simulink model "DWPUSH"  (R2026b)
settings: Solver=VariableStepAuto
undefined symbols (not defined in the file): Ac, Af, Ar, InitLinkage, Left, Linkage, Visual, X, Y, Z
libraries: sm_lib x57, Suspension_Utilities x43, nesl_utility x12, Linkage_Shock x1, fl_lib x1
(part 2 of 4)

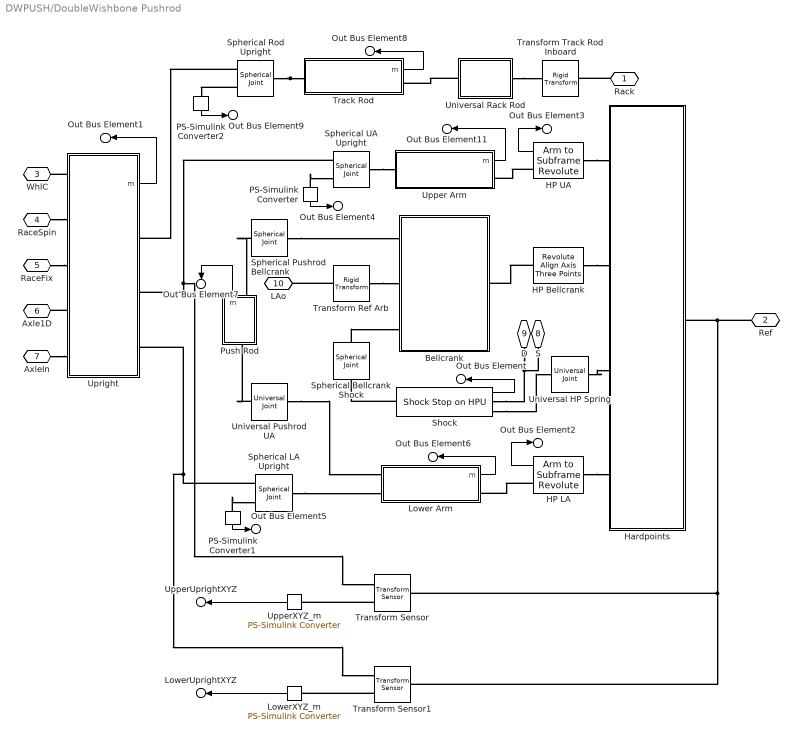
== system DWPUSH/DoubleWishbone Pushrod ==
  Bellcrank : Subsystem  mask(Bellcrank){popup_leftRight=Left, hp_bcr_pivot=hp_bcr_pivot, hp_bcr_shock=hp_spr_bcr, hp_rod=hp_pushrod_in, hp_arb=hp_arb, bcr_mass=bcr_mass, clr_bcr=clr_bcr, opc_bcr=opc_bcr, radius_bcr=radius_bcr}
      mask prompts: popup_leftRight "Left/Right"; hp_bcr_pivot "HP Bellcrank Pivot [xyz] (m)"; hp_bcr_shock "HP Bellcrank Shock [xyz] (m)"; hp_rod "HP Bellcrank Rod [xyz] (m)"; hp_arb "HP Bellcrank ARB [xyz] (m)"; bcr_mass "Mass (kg)"; clr_bcr "Color [RGB]"; opc_bcr "Opacity (0-1)"; radius_bcr "Radius (m)"
      mask help: Models a bellcrank with one pivot and 3 attachment points. The axis of the pivot is normal to the plane formed by the pivot, connection to the rod, and connection to the shock.
      mask init:
      | if(popup_leftRight == 1)
      |     rhs_susp = 1;
      | elseif(popup_leftRight == 2)
      |     rhs_susp = -1;
      | end
      | 
      | rhs_hp = [1 rhs_susp 1];
      mask TypeOptions popup_leftRight: Left | Right
      mask TypeOptions clr_bcr: Arm Pivot ARB/clr_solid | Arm Pivot Rod/clr_solid | Arm Pivot Shock/clr_solid | Arm Rod Shock/clr_solid
      mask TypeOptions opc_bcr: Arm Pivot ARB/opc_solid | Arm Pivot Rod/opc_solid | Arm Pivot Shock/opc_solid | Arm Rod Shock/opc_solid
      mask TypeOptions radius_bcr: Arm Pivot ARB/rad_solid | Arm Pivot Rod/rad_solid | Arm Pivot Shock/rad_solid | Arm Rod Shock/rad_solid
      mask DialogControl cont_ua Prompt: UA
      mask DialogControl cont_vis_ua Prompt: Visualization
      mask Display: image('sm_car_vehicle_linkage_bellcrank_IMAGE.png');
  HP Bellcrank : Suspension_Utilities/Revolute Align Axis Three Points  popup_leftRight=Left  hp_1=hp_bcr_pivot  hp_2=hp_pushrod_in  hp_3=hp_spr_bcr  positionTargetSpecify=off  PositionTargetValue=0
      settings: SourceProductName=SmCar - Suspension Utilites
  HP LA : Suspension_Utilities/Arm to Subframe Revolute  VariantControl=Variant1  LabelModeActiveChoice=Bushing_AxRad  popup_leftRight=Left  hp_f=hp_in_f_ua  hp_r=hp_in_r_ua  Connection=Lower_Arm_to_Subframe  VariantLabel=Lower_Arm_to_Subframe.class.Value
      settings: AttributesFormatString=%<ActiveVariant>  SourceProductName=SmCar - Suspension Utilites
  HP UA : Suspension_Utilities/Arm to Subframe Revolute  VariantControl=Variant1  LabelModeActiveChoice=Bushing_AxRad  popup_leftRight=Left  hp_f=hp_in_f_ua  hp_r=hp_in_r_ua  Connection=Upper_Arm_to_Subframe  VariantLabel=Upper_Arm_to_Subframe.class.Value
      settings: AttributesFormatString=%<ActiveVariant>  SourceProductName=SmCar - Suspension Utilites
  Hardpoints : Subsystem  mask{popup_leftRight=Left, hp_in_f_ua=hp_in_f_ua, hp_in_r_ua=hp_in_r_ua, hp_in_f_la=hp_in_f_la, hp_in_r_la=hp_in_r_la, hp_bellcrank=hp_bcr_pivot, hp_spr_top=hp_spr_body, clr_hp=clr_hp, opc_hp=opc_hp, size_hp=size_hp}
      mask prompts: popup_leftRight "Left/Right"; hp_in_f_ua "Upper Arm Front [xyz] (m)"; hp_in_r_ua "Upper Arm Rear [xyz] (m)"; hp_in_f_la "Lower Arm Front [xyz] (m)"; hp_in_r_la "Lower Arm Rear [xyz] (m)"; hp_bellcrank "Bellcrank Pivot [xyz] (m)"; hp_spr_top "Spring [xyz] (m)"
      mask init:
      | % Set parameter for mirroring (+y or -y)
      | if(popup_leftRight == 1)
      |     rhs_susp = 1;    
      | elseif(popup_leftRight == 2)
      |     rhs_susp = -1;
      | end
      | 
      | rhs_hp = [1 rhs_susp 1];
      mask TypeOptions popup_leftRight: Left | Right
      mask TypeOptions clr_hp: Subsystem/Vis HP LAf/GraphicDiffuseColor | Vis HP LAr/GraphicDiffuseColor | Vis HP Spring/GraphicDiffuseColor | Vis HP UAf/GraphicDiffuseColor | Vis HP UAr/GraphicDiffuseColor
      mask TypeOptions opc_hp: Subsystem/Vis HP LAf/GraphicOpacity | Vis HP LAr/GraphicOpacity | Vis HP Spring/GraphicOpacity | Vis HP UAf/GraphicOpacity | Vis HP UAr/GraphicOpacity
      mask DialogControl cont_hp Prompt: Hardpoints
      mask DialogControl cont_vis_hp Prompt: Visualization
      mask DialogControl text_clr_hp Prompt: Color [RGB]
      mask DialogControl text_opc_hp Prompt: Opac. (0-1)
      mask DialogControl text_size_hp Prompt: Size (m)
      mask DialogControl text_hp Prompt: Hardpoints
      mask Display: image('sm_car_vehicle_linkage_dw_pullrod_hp_IMAGE.png');
  Lower Arm : Subsystem  mask(Lower Arm (Wishbone)){popup_leftRight=Left, hp_in_f=hp_in_f_la, hp_in_r=hp_in_r_la, hp_out=hp_out_la, hp_rod=hp_pushrod_out, la_mass=la_mass, clr_solid=clr_la, opc_solid=opc_la, rad_solid=radius_la}
      mask prompts: popup_leftRight "Left/Right"; hp_in_f "Inboard Front [xyz] (m)"; hp_in_r "Inboard Rear [xyz] (m)"; hp_out "Outboard [xyz] (m)"; hp_rod "Rod [xyz] (m)"; la_mass "Mass (kg)"; clr_solid "Color [RGB]"; opc_solid "Opacity (0-1)"; rad_solid "Radius (m)"
      mask help: This subsystem models the lower arm of a wishbone suspension. It can be configured to have one or two attachment points to the chassis. There are connections to the upright and spring.
      mask init:
      | % Set parameter for mirroring (+y or -y)
      | if(popup_leftRight == 1)
      |     rhs_susp = 1;
      | elseif(popup_leftRight == 2)
      |     rhs_susp = -1;
      | end
      | 
      | rhs_hp = [1 rhs_susp 1];
      | 
      | 
      |     hp_rod_f=hp_out-(hp_out-hp_in_f)/2;
      |     hp_rod_r=hp_out-(hp_out-hp_in_r)/2;
      mask Help: web ('sm_car_lower_arm_help.html')
      mask TypeOptions popup_leftRight: Left | Right
      mask TypeOptions clr_solid: Arm F1/clr_solid | Arm F2/clr_solid | Arm R1/clr_solid | Arm R2/clr_solid
      mask TypeOptions opc_solid: Arm F1/opc_solid | Arm F2/opc_solid | Arm R1/opc_solid | Arm R2/opc_solid
      mask TypeOptions rad_solid: Arm F1/rad_solid | Arm F2/rad_solid | Arm R1/rad_solid | Arm R2/rad_solid
      mask DialogControl cont_ua Prompt: LA
      mask DialogControl cont_vis_la Prompt: Visualization
      mask Display: image('sm_car_vehicle_linkage_dw_ua_IMAGE.png');
  LowerXYZ_m : nesl_utility/PS-Simulink Converter  PhysicalDomain=network_engine_domain  SubClassName=ps_output  LeftPortType=input  RightPortType=output  PseudoPeriodic=off  Frequencies=[]  VectorFormat=inherit  Unit=m  AffineConversion=off
  PS-Simulink Converter : nesl_utility/PS-Simulink Converter  PhysicalDomain=network_engine_domain  SubClassName=ps_output  LeftPortType=input  RightPortType=output  PseudoPeriodic=off  Frequencies=[]  VectorFormat=inherit  Unit=inherit  AffineConversion=off
  PS-Simulink Converter1 : nesl_utility/PS-Simulink Converter  PhysicalDomain=network_engine_domain  SubClassName=ps_output  LeftPortType=input  RightPortType=output  PseudoPeriodic=off  Frequencies=[]  VectorFormat=inherit  Unit=inherit  AffineConversion=off
  PS-Simulink Converter2 : nesl_utility/PS-Simulink Converter  PhysicalDomain=network_engine_domain  SubClassName=ps_output  LeftPortType=input  RightPortType=output  PseudoPeriodic=off  Frequencies=[]  VectorFormat=inherit  Unit=inherit  AffineConversion=off
  Push Rod : Subsystem  VariantControl=Steer  mask(Rod){popup_leftRight=Left, hp_in=hp_pushrod_in, hp_out=hp_pushrod_out, rod_mass=pullrod_mass, clr_conn_rod=clr_conn_pullrod, opc_conn_rod=opc_conn_pullrod, size_conn_rod=size_conn_pullrod, clr_rod=clr_pullrod, opc_rod=opc_pullrod, radius_rod=radius_pullrod}
      mask prompts: popup_leftRight "Left/Right"; hp_in "Bellcrank [xyz] (m)"; hp_out "Upper Arm [xyz] (m)"; rod_mass "Mass (Kg)"
      mask help: Rod connecting two hard points
      mask init:
      | if(popup_leftRight == 1)
      |     rhs_rod = 1;
      | elseif(popup_leftRight == 2)
      |     rhs_rod = -1;
      | end
      | rhs_hp=[1 rhs_rod 1];
      | 
      |     hp_rod_c=hp_out-(hp_out-hp_in)/2;
      mask TypeOptions popup_leftRight: Left | Right
      mask TypeOptions clr_conn_rod:
      | Vis
      | Rod
      | Out/GraphicDiffuseColor | Vis
      | Rod
      | In/GraphicDiffuseColor
      mask TypeOptions opc_conn_rod:
      | Vis
      | Rod
      | Out/GraphicOpacity | Vis
      | Rod
      | In/GraphicOpacity
      mask TypeOptions clr_rod: Rod/clr_solid
      mask TypeOptions opc_rod: Rod/opc_solid
      mask TypeOptions radius_rod: Rod/rad_solid
      mask DialogControl cont_rod Prompt: Rod
      mask DialogControl grp_rod Prompt: Rod
      mask DialogControl cont_vis_rod Prompt: Visualization
      mask DialogControl text_clr_rod Prompt: Color [RGB]
      mask DialogControl text_opc_rod Prompt: Opac. (0-1)
      mask DialogControl text_size_rod Prompt: Size (m)
      mask DialogControl text_conn_rod Prompt: Connections
      mask DialogControl text_rod_rod Prompt: Rod
      mask Display: image('sm_car_vehicle_linkage_pushrod_IMAGE.png');
  Shock : Linkage_Shock/Shock Stop on HPU  shock_pist_mass=shock_pist_mass  shock_cyl_mass=shock_cyl_mass  hp_spr_top=hp_spr_body  hp_spr_bot=hp_spr_bcr  up_lim_bumpstop=up_lim_bumpstop  low_lim_bumpstop=low_lim_bumpstop  clr_conn_shock=clr_conn_shock  opc_conn_shock=opc_conn_shock  size_conn_shock=size_conn_shock  clr_shock_cyl=clr_shock_cyl  opc_shock_cyl=opc_shock_cyl  radius_shock_cyl=radius_shock_cyl  clr_shock_piston=clr_shock_piston  opc_shock_piston=opc_shock_piston  clr_shock_bumpstop=clr_shock_bumpstop  opc_shock_bumpstop=opc_shock_bumpstop  deadvol_len_shock_cyl=deadvol_len_shock_cyl  piston_len_shock=piston_len_shock  cyl_cap_len_shock=cyl_cap_len_shock  bumpstop_len_shock=bumpstop_len_shock
  Spherical Bellcrank Shock : sm_lib/Joints/Spherical Joint  JointMode=Normal  CompositeWrenchDir=FollowerOnBase  CompositeWrenchFrame=BaseFrame  SenseConstraintForce=off  SenseConstraintTorque=off  SenseTotalForce=off  SenseTotalTorque=off  PositionTargetSpecify=off  PositionTargetPriority=High  PositionTargetRotationMethod=None  PositionTargetFollAlignAxisA=+X  PositionTargetBaseAlignAxisA=+Y  PositionTargetFollAlignAxisB=+Y  PositionTargetBaseAlignAxisB=+Z  PositionTargetRotationStandardAxis=+Z  PositionTargetRotationAngle=0.0  PositionTargetRotationAngleUnits=deg  PositionTargetRotationArbitraryAxis=[0 0 1]  PositionTargetRotationSequenceAxes=FollowerAxes  PositionTargetRotationSequence=XYX  PositionTargetRotationSequenceAngles=[0 0 0]  PositionTargetRotationSequenceAnglesUnits=deg  PositionTargetRotationMatrix=[1 0 0; 0 1 0; 0 0 1]  PositionTargetQuaternion=[1 0 0 0]  VelocityTargetSpecify=off  VelocityTargetPriority=High  VelocityTargetValue=[0 0 0]  VelocityTargetValueUnits=deg/s  VelocityTargetInFollowerFrame=on  EqPosRotationMethod=None  EqPosFollAlignAxisA=+X  EqPosBaseAlignAxisA=+Y  EqPosFollAlignAxisB=+Y  EqPosBaseAlignAxisB=+Z  EqPosRotationStandardAxis=+Z  EqPosRotationAngle=0.0  EqPosRotationAngleUnits=deg  EqPosRotationArbitraryAxis=[0 0 1]  EqPosRotationSequenceAxes=FollowerAxes  EqPosRotationSequence=XYX  EqPosRotationSequenceAngles=[0 0 0]  EqPosRotationSequenceAnglesUnits=deg  EqPosRotationMatrix=[1 0 0; 0 1 0; 0 0 1]  EqPosQuaternion=[1 0 0 0]  SpringStiffness=0  SpringStiffnessUnits=N*m/deg  DampingCoefficient=0  DampingCoefficientUnits=N*m/(deg/s)  LowerLimitSpecify=off  LowerLimitBound=15  LowerLimitBoundUnits=deg  LowerLimitStiffness=1e4  LowerLimitStiffnessUnits=N*m/deg  LowerLimitDamping=10  LowerLimitDampingUnits=N*m/(deg/s)  LowerLimitTransitionRegionWidth=0.1  LowerLimitTransitionRegionWidthUnits=deg  UpperLimitSpecify=off  UpperLimitBound=45  UpperLimitBoundUnits=deg  UpperLimitStiffness=1e4  UpperLimitStiffnessUnits=N*m/deg  UpperLimitDamping=10  UpperLimitDampingUnits=N*m/(deg/s)  UpperLimitTransitionRegionWidth=0.1  UpperLimitTransitionRegionWidthUnits=deg  TorqueActuationMode=NoTorque  ActuateTorqueX=off  ActuateTorqueY=off  ActuateTorqueZ=off  ActuateTorque=off  ActuationFrame=BaseFrame  SensePosition=off  SenseVelocityX=off  SenseVelocityY=off  SenseVelocityZ=off  SenseVelocity=off  SenseAccelerationX=off  SenseAccelerationY=off  SenseAccelerationZ=off  SenseAcceleration=off  SenseLowerLimitTorqueMag=off  SenseUpperLimitTorqueMag=off  SensingFrame=BaseFrame
  Spherical LA Upright : sm_lib/Joints/Spherical Joint  JointMode=Normal  CompositeWrenchDir=FollowerOnBase  CompositeWrenchFrame=BaseFrame  SenseConstraintForce=off  SenseConstraintTorque=off  SenseTotalForce=on  SenseTotalTorque=off  PositionTargetSpecify=off  PositionTargetPriority=High  PositionTargetRotationMethod=None  PositionTargetFollAlignAxisA=+X  PositionTargetBaseAlignAxisA=+Y  PositionTargetFollAlignAxisB=+Y  PositionTargetBaseAlignAxisB=+Z  PositionTargetRotationStandardAxis=+Z  PositionTargetRotationAngle=0.0  PositionTargetRotationAngleUnits=deg  PositionTargetRotationArbitraryAxis=[0 0 1]  PositionTargetRotationSequenceAxes=FollowerAxes  PositionTargetRotationSequence=XYX  PositionTargetRotationSequenceAngles=[0 0 0]  PositionTargetRotationSequenceAnglesUnits=deg  PositionTargetRotationMatrix=[1 0 0; 0 1 0; 0 0 1]  PositionTargetQuaternion=[1 0 0 0]  VelocityTargetSpecify=off  VelocityTargetPriority=High  VelocityTargetValue=[0 0 0]  VelocityTargetValueUnits=deg/s  VelocityTargetInFollowerFrame=on  EqPosRotationMethod=None  EqPosFollAlignAxisA=+X  EqPosBaseAlignAxisA=+Y  EqPosFollAlignAxisB=+Y  EqPosBaseAlignAxisB=+Z  EqPosRotationStandardAxis=+Z  EqPosRotationAngle=0.0  EqPosRotationAngleUnits=deg  EqPosRotationArbitraryAxis=[0 0 1]  EqPosRotationSequenceAxes=FollowerAxes  EqPosRotationSequence=XYX  EqPosRotationSequenceAngles=[0 0 0]  EqPosRotationSequenceAnglesUnits=deg  EqPosRotationMatrix=[1 0 0; 0 1 0; 0 0 1]  EqPosQuaternion=[1 0 0 0]  SpringStiffness=0  SpringStiffnessUnits=N*m/deg  DampingCoefficient=0  DampingCoefficientUnits=N*m/(deg/s)  LowerLimitSpecify=off  LowerLimitBound=15  LowerLimitBoundUnits=deg  LowerLimitStiffness=1e4  LowerLimitStiffnessUnits=N*m/deg  LowerLimitDamping=10  LowerLimitDampingUnits=N*m/(deg/s)  LowerLimitTransitionRegionWidth=0.1  LowerLimitTransitionRegionWidthUnits=deg  UpperLimitSpecify=off  UpperLimitBound=45  UpperLimitBoundUnits=deg  UpperLimitStiffness=1e4  UpperLimitStiffnessUnits=N*m/deg  UpperLimitDamping=10  UpperLimitDampingUnits=N*m/(deg/s)  UpperLimitTransitionRegionWidth=0.1  UpperLimitTransitionRegionWidthUnits=deg  TorqueActuationMode=NoTorque  ActuateTorqueX=off  ActuateTorqueY=off  ActuateTorqueZ=off  ActuateTorque=off  ActuationFrame=BaseFrame  SensePosition=off  SenseVelocityX=off  SenseVelocityY=off  SenseVelocityZ=off  SenseVelocity=off  SenseAccelerationX=off  SenseAccelerationY=off  SenseAccelerationZ=off  SenseAcceleration=off  SenseLowerLimitTorqueMag=off  SenseUpperLimitTorqueMag=off  SensingFrame=BaseFrame
  Spherical Pushrod Bellcrank : sm_lib/Joints/Spherical Joint  JointMode=Normal  CompositeWrenchDir=FollowerOnBase  CompositeWrenchFrame=BaseFrame  SenseConstraintForce=off  SenseConstraintTorque=off  SenseTotalForce=off  SenseTotalTorque=off  PositionTargetSpecify=off  PositionTargetPriority=High  PositionTargetRotationMethod=None  PositionTargetFollAlignAxisA=+X  PositionTargetBaseAlignAxisA=+Y  PositionTargetFollAlignAxisB=+Y  PositionTargetBaseAlignAxisB=+Z  PositionTargetRotationStandardAxis=+Z  PositionTargetRotationAngle=0.0  PositionTargetRotationAngleUnits=deg  PositionTargetRotationArbitraryAxis=[0 0 1]  PositionTargetRotationSequenceAxes=FollowerAxes  PositionTargetRotationSequence=XYX  PositionTargetRotationSequenceAngles=[0 0 0]  PositionTargetRotationSequenceAnglesUnits=deg  PositionTargetRotationMatrix=[1 0 0; 0 1 0; 0 0 1]  PositionTargetQuaternion=[1 0 0 0]  VelocityTargetSpecify=off  VelocityTargetPriority=High  VelocityTargetValue=[0 0 0]  VelocityTargetValueUnits=deg/s  VelocityTargetInFollowerFrame=on  EqPosRotationMethod=None  EqPosFollAlignAxisA=+X  EqPosBaseAlignAxisA=+Y  EqPosFollAlignAxisB=+Y  EqPosBaseAlignAxisB=+Z  EqPosRotationStandardAxis=+Z  EqPosRotationAngle=0.0  EqPosRotationAngleUnits=deg  EqPosRotationArbitraryAxis=[0 0 1]  EqPosRotationSequenceAxes=FollowerAxes  EqPosRotationSequence=XYX  EqPosRotationSequenceAngles=[0 0 0]  EqPosRotationSequenceAnglesUnits=deg  EqPosRotationMatrix=[1 0 0; 0 1 0; 0 0 1]  EqPosQuaternion=[1 0 0 0]  SpringStiffness=0  SpringStiffnessUnits=N*m/deg  DampingCoefficient=0  DampingCoefficientUnits=N*m/(deg/s)  LowerLimitSpecify=off  LowerLimitBound=15  LowerLimitBoundUnits=deg  LowerLimitStiffness=1e4  LowerLimitStiffnessUnits=N*m/deg  LowerLimitDamping=10  LowerLimitDampingUnits=N*m/(deg/s)  LowerLimitTransitionRegionWidth=0.1  LowerLimitTransitionRegionWidthUnits=deg  UpperLimitSpecify=off  UpperLimitBound=45  UpperLimitBoundUnits=deg  UpperLimitStiffness=1e4  UpperLimitStiffnessUnits=N*m/deg  UpperLimitDamping=10  UpperLimitDampingUnits=N*m/(deg/s)  UpperLimitTransitionRegionWidth=0.1  UpperLimitTransitionRegionWidthUnits=deg  TorqueActuationMode=NoTorque  ActuateTorqueX=off  ActuateTorqueY=off  ActuateTorqueZ=off  ActuateTorque=off  ActuationFrame=BaseFrame  SensePosition=off  SenseVelocityX=off  SenseVelocityY=off  SenseVelocityZ=off  SenseVelocity=off  SenseAccelerationX=off  SenseAccelerationY=off  SenseAccelerationZ=off  SenseAcceleration=off  SenseLowerLimitTorqueMag=off  SenseUpperLimitTorqueMag=off  SensingFrame=BaseFrame
  Spherical Rod Upright : sm_lib/Joints/Spherical Joint  JointMode=Normal  CompositeWrenchDir=FollowerOnBase  CompositeWrenchFrame=BaseFrame  SenseConstraintForce=off  SenseConstraintTorque=off  SenseTotalForce=on  SenseTotalTorque=off  PositionTargetSpecify=off  PositionTargetPriority=High  PositionTargetRotationMethod=None  PositionTargetFollAlignAxisA=+X  PositionTargetBaseAlignAxisA=+Y  PositionTargetFollAlignAxisB=+Y  PositionTargetBaseAlignAxisB=+Z  PositionTargetRotationStandardAxis=+Z  PositionTargetRotationAngle=0.0  PositionTargetRotationAngleUnits=deg  PositionTargetRotationArbitraryAxis=[0 0 1]  PositionTargetRotationSequenceAxes=FollowerAxes  PositionTargetRotationSequence=XYX  PositionTargetRotationSequenceAngles=[0 0 0]  PositionTargetRotationSequenceAnglesUnits=deg  PositionTargetRotationMatrix=[1 0 0; 0 1 0; 0 0 1]  PositionTargetQuaternion=[1 0 0 0]  VelocityTargetSpecify=off  VelocityTargetPriority=High  VelocityTargetValue=[0 0 0]  VelocityTargetValueUnits=deg/s  VelocityTargetInFollowerFrame=on  EqPosRotationMethod=None  EqPosFollAlignAxisA=+X  EqPosBaseAlignAxisA=+Y  EqPosFollAlignAxisB=+Y  EqPosBaseAlignAxisB=+Z  EqPosRotationStandardAxis=+Z  EqPosRotationAngle=0.0  EqPosRotationAngleUnits=deg  EqPosRotationArbitraryAxis=[0 0 1]  EqPosRotationSequenceAxes=FollowerAxes  EqPosRotationSequence=XYX  EqPosRotationSequenceAngles=[0 0 0]  EqPosRotationSequenceAnglesUnits=deg  EqPosRotationMatrix=[1 0 0; 0 1 0; 0 0 1]  EqPosQuaternion=[1 0 0 0]  SpringStiffness=0  SpringStiffnessUnits=N*m/deg  DampingCoefficient=0  DampingCoefficientUnits=N*m/(deg/s)  LowerLimitSpecify=off  LowerLimitBound=15  LowerLimitBoundUnits=deg  LowerLimitStiffness=1e4  LowerLimitStiffnessUnits=N*m/deg  LowerLimitDamping=10  LowerLimitDampingUnits=N*m/(deg/s)  LowerLimitTransitionRegionWidth=0.1  LowerLimitTransitionRegionWidthUnits=deg  UpperLimitSpecify=off  UpperLimitBound=45  UpperLimitBoundUnits=deg  UpperLimitStiffness=1e4  UpperLimitStiffnessUnits=N*m/deg  UpperLimitDamping=10  UpperLimitDampingUnits=N*m/(deg/s)  UpperLimitTransitionRegionWidth=0.1  UpperLimitTransitionRegionWidthUnits=deg  TorqueActuationMode=NoTorque  ActuateTorqueX=off  ActuateTorqueY=off  ActuateTorqueZ=off  ActuateTorque=off  ActuationFrame=BaseFrame  SensePosition=off  SenseVelocityX=off  SenseVelocityY=off  SenseVelocityZ=off  SenseVelocity=off  SenseAccelerationX=off  SenseAccelerationY=off  SenseAccelerationZ=off  SenseAcceleration=off  SenseLowerLimitTorqueMag=off  SenseUpperLimitTorqueMag=off  SensingFrame=BaseFrame
  Spherical UA Upright : sm_lib/Joints/Spherical Joint  JointMode=Normal  CompositeWrenchDir=FollowerOnBase  CompositeWrenchFrame=BaseFrame  SenseConstraintForce=off  SenseConstraintTorque=off  SenseTotalForce=on  SenseTotalTorque=off  PositionTargetSpecify=on  PositionTargetPriority=High  PositionTargetRotationMethod=StandardAxis  PositionTargetFollAlignAxisA=+X  PositionTargetBaseAlignAxisA=+Y  PositionTargetFollAlignAxisB=+Y  PositionTargetBaseAlignAxisB=+Z  PositionTargetRotationStandardAxis=+Z  PositionTargetRotationAngle=0.0  PositionTargetRotationAngleUnits=deg  PositionTargetRotationArbitraryAxis=[0 0 1]  PositionTargetRotationSequenceAxes=FollowerAxes  PositionTargetRotationSequence=XYX  PositionTargetRotationSequenceAngles=[0 0 0]  PositionTargetRotationSequenceAnglesUnits=deg  PositionTargetRotationMatrix=[1 0 0; 0 1 0; 0 0 1]  PositionTargetQuaternion=[1 0 0 0]  VelocityTargetSpecify=off  VelocityTargetPriority=High  VelocityTargetValue=[0 0 0]  VelocityTargetValueUnits=deg/s  VelocityTargetInFollowerFrame=on  EqPosRotationMethod=None  EqPosFollAlignAxisA=+X  EqPosBaseAlignAxisA=+Y  EqPosFollAlignAxisB=+Y  EqPosBaseAlignAxisB=+Z  EqPosRotationStandardAxis=+Z  EqPosRotationAngle=0.0  EqPosRotationAngleUnits=deg  EqPosRotationArbitraryAxis=[0 0 1]  EqPosRotationSequenceAxes=FollowerAxes  EqPosRotationSequence=XYX  EqPosRotationSequenceAngles=[0 0 0]  EqPosRotationSequenceAnglesUnits=deg  EqPosRotationMatrix=[1 0 0; 0 1 0; 0 0 1]  EqPosQuaternion=[1 0 0 0]  SpringStiffness=0  SpringStiffnessUnits=N*m/deg  DampingCoefficient=0  DampingCoefficientUnits=N*m/(deg/s)  LowerLimitSpecify=off  LowerLimitBound=15  LowerLimitBoundUnits=deg  LowerLimitStiffness=1e4  LowerLimitStiffnessUnits=N*m/deg  LowerLimitDamping=10  LowerLimitDampingUnits=N*m/(deg/s)  LowerLimitTransitionRegionWidth=0.1  LowerLimitTransitionRegionWidthUnits=deg  UpperLimitSpecify=off  UpperLimitBound=45  UpperLimitBoundUnits=deg  UpperLimitStiffness=1e4  UpperLimitStiffnessUnits=N*m/deg  UpperLimitDamping=10  UpperLimitDampingUnits=N*m/(deg/s)  UpperLimitTransitionRegionWidth=0.1  UpperLimitTransitionRegionWidthUnits=deg  TorqueActuationMode=NoTorque  ActuateTorqueX=off  ActuateTorqueY=off  ActuateTorqueZ=off  ActuateTorque=off  ActuationFrame=BaseFrame  SensePosition=off  SenseVelocityX=off  SenseVelocityY=off  SenseVelocityZ=off  SenseVelocity=off  SenseAccelerationX=off  SenseAccelerationY=off  SenseAccelerationZ=off  SenseAcceleration=off  SenseLowerLimitTorqueMag=off  SenseUpperLimitTorqueMag=off  SensingFrame=FollowerFrame
  Track Rod : Subsystem  VariantControl=Steer  mask(Rod){popup_leftRight=Left, hp_in=hp_in_rod, hp_out=hp_upr_rod, rod_mass=rod_mass, clr_conn_rod=clr_conn_rod, opc_conn_rod=opc_conn_rod, size_conn_rod=size_conn_rod, clr_rod=clr_rod, opc_rod=opc_rod, radius_rod=radius_rod}
      mask prompts: popup_leftRight "Left/Right"; hp_in "Inboard [xyz] (m)"; hp_out "Outboard [xyz] (m)"; rod_mass "Mass (kg)"
      mask help: Rod connecting two hard points
      mask init:
      | if(popup_leftRight == 1)
      |     rhs_rod = 1;
      | elseif(popup_leftRight == 2)
      |     rhs_rod = -1;
      | end
      | rhs_hp=[1 rhs_rod 1];
      | hp_rod_c=hp_out-(hp_out-hp_in)/2;
      mask TypeOptions popup_leftRight: Left | Right
      mask TypeOptions rod_mass: Rod/Mass
      mask TypeOptions clr_conn_rod:
      | Vis
      | Upright
      | Steer/GraphicDiffuseColor | Vis
      | Rack
      | Rod/GraphicDiffuseColor
      mask TypeOptions opc_conn_rod:
      | Vis
      | Upright
      | Steer/GraphicOpacity | Vis
      | Rack
      | Rod/GraphicOpacity
      mask TypeOptions clr_rod: Rod/clr_solid
      mask TypeOptions opc_rod: Rod/opc_solid
      mask TypeOptions radius_rod: Rod/rad_solid
      mask DialogControl cont_rod Prompt: Rod
      mask DialogControl grp_rod Prompt: Rod
      mask DialogControl cont_vis_rod Prompt: Visualization
      mask DialogControl text_clr_rod Prompt: Color [RGB]
      mask DialogControl text_opc_rod Prompt: Opac. (0-1)
      mask DialogControl text_size_rod Prompt: Size (m)
      mask DialogControl text_conn_rod Prompt: Connections
      mask DialogControl text_rod_rod Prompt: Rod
      mask Display: image('sm_car_linkage_trackrod_IMAGE.png');
  Transform Ref Arb : sm_lib/Frames and Transforms/Rigid Transform  RotationMethod=None  FollAlignAxisA=+X  BaseAlignAxisA=+Y  FollAlignAxisB=+Y  BaseAlignAxisB=+Z  RotationStandardAxis=+Z  RotationAngle=0.0  RotationAngleUnits=deg  RotationArbitraryAxis=[0 0 1]  RotationSequenceAxes=FollowerAxes  RotationSequence=XYX  RotationSequenceAngles=[0 0 0]  RotationSequenceAnglesUnits=deg  RotationMatrix=[1 0 0; 0 1 0; 0 0 1]  Quaternion=[1 0 0 0]  TranslationMethod=Cartesian  TranslationCartesianOffset=hp_arb.*[1 rhs_susp 1]  TranslationCartesianOffsetUnits=m  TranslationStandardAxis=+Z  TranslationStandardOffset=0  TranslationStandardOffsetUnits=m  TranslationROffset=0  TranslationROffsetUnits=m  TranslationThetaOffset=0  TranslationThetaOffsetUnits=deg  TranslationZOffset=0  TranslationZOffsetUnits=m
  Transform Sensor : sm_lib/Frames and Transforms/Transform Sensor  ObservationFrame=Base  ExpressedInFrame=Base  RotationSequence=XYX  SenseAngle=off  SenseAxis=off  SenseQ=off  SenseR=off  SenseRotationSequence=off  SenseOmegaX=off  SenseOmegaY=off  SenseOmegaZ=off  SenseOmega=off  SenseQDot=off  SenseRDot=off  SenseRotationSequenceDot=off  SenseAlphaX=off  SenseAlphaY=off  SenseAlphaZ=off  SenseAlpha=off  SenseQDDot=off  SenseRDDot=off  SenseX=off  SenseY=off  SenseZ=off  SenseXYZ=on  SenseRad=off  SenseAzim=off  SenseDist=off  SenseInc=off  SenseXDot=off  SenseYDot=off  SenseZDot=off  SenseXYZDot=off  SenseRadDot=off  SenseAzimDot=off  SenseDistDot=off  SenseIncDot=off  SenseXDDot=off  SenseYDDot=off  SenseZDDot=off  SenseXYZDDot=off  SenseRadDDot=off  SenseAzimDDot=off  SenseDistDDot=off  SenseIncDDot=off
  Transform Sensor1 : sm_lib/Frames and Transforms/Transform Sensor  ObservationFrame=Base  ExpressedInFrame=Base  RotationSequence=XYX  SenseAngle=off  SenseAxis=off  SenseQ=off  SenseR=off  SenseRotationSequence=off  SenseOmegaX=off  SenseOmegaY=off  SenseOmegaZ=off  SenseOmega=off  SenseQDot=off  SenseRDot=off  SenseRotationSequenceDot=off  SenseAlphaX=off  SenseAlphaY=off  SenseAlphaZ=off  SenseAlpha=off  SenseQDDot=off  SenseRDDot=off  SenseX=off  SenseY=off  SenseZ=off  SenseXYZ=on  SenseRad=off  SenseAzim=off  SenseDist=off  SenseInc=off  SenseXDot=off  SenseYDot=off  SenseZDot=off  SenseXYZDot=off  SenseRadDot=off  SenseAzimDot=off  SenseDistDot=off  SenseIncDot=off  SenseXDDot=off  SenseYDDot=off  SenseZDDot=off  SenseXYZDDot=off  SenseRadDDot=off  SenseAzimDDot=off  SenseDistDDot=off  SenseIncDDot=off
  Transform Track Rod Inboard : sm_lib/Frames and Transforms/Rigid Transform  RotationMethod=None  FollAlignAxisA=+X  BaseAlignAxisA=+Y  FollAlignAxisB=+Y  BaseAlignAxisB=+Z  RotationStandardAxis=+Z  RotationAngle=0.0  RotationAngleUnits=deg  RotationArbitraryAxis=[0 0 1]  RotationSequenceAxes=FollowerAxes  RotationSequence=XYX  RotationSequenceAngles=[0 0 0]  RotationSequenceAnglesUnits=deg  RotationMatrix=[1 0 0; 0 1 0; 0 0 1]  Quaternion=[1 0 0 0]  TranslationMethod=Cartesian  TranslationCartesianOffset=hp_in_rod.*[1 rhs_susp 1]  TranslationCartesianOffsetUnits=m  TranslationStandardAxis=+Z  TranslationStandardOffset=0  TranslationStandardOffsetUnits=m  TranslationROffset=0  TranslationROffsetUnits=m  TranslationThetaOffset=0  TranslationThetaOffsetUnits=deg  TranslationZOffset=0  TranslationZOffsetUnits=m
  Universal HP Spring : sm_lib/Joints/Universal Joint  JointMode=Normal  CompositeWrenchDir=FollowerOnBase  CompositeWrenchFrame=BaseFrame  SenseConstraintForce=off  SenseConstraintTorque=off  SenseTotalForce=off  SenseTotalTorque=off  RxPositionTargetSpecify=off  RxPositionTargetPriority=High  RxPositionTargetValue=0  RxPositionTargetValueUnits=deg  RxVelocityTargetSpecify=off  RxVelocityTargetPriority=High  RxVelocityTargetValue=0  RxVelocityTargetValueUnits=deg/s  RxEquilibriumPosition=0  RxEquilibriumPositionUnits=deg  RxSpringStiffness=0  RxSpringStiffnessUnits=N*m/deg  RxDampingCoefficient=0  RxDampingCoefficientUnits=N*m/(deg/s)  RxLowerLimitSpecify=off  RxLowerLimitBound=-90  RxLowerLimitBoundUnits=deg  RxLowerLimitStiffness=1e4  RxLowerLimitStiffnessUnits=N*m/deg  RxLowerLimitDamping=10  RxLowerLimitDampingUnits=N*m/(deg/s)  RxLowerLimitTransitionRegionWidth=0.1  RxLowerLimitTransitionRegionWidthUnits=deg  RxUpperLimitSpecify=off  RxUpperLimitBound=90  RxUpperLimitBoundUnits=deg  RxUpperLimitStiffness=1e4  RxUpperLimitStiffnessUnits=N*m/deg  RxUpperLimitDamping=10  RxUpperLimitDampingUnits=N*m/(deg/s)  RxUpperLimitTransitionRegionWidth=0.1  RxUpperLimitTransitionRegionWidthUnits=deg  RxTorqueActuationMode=NoTorque  RxMotionActuationMode=ComputedMotion  RxSensePosition=off  RxSenseVelocity=off  RxSenseAcceleration=off  RxSenseTorqueForce=off  RxSenseLowerLimitTorqueForce=off  RxSenseUpperLimitTorqueForce=off  RyPositionTargetSpecify=off  RyPositionTargetPriority=High  RyPositionTargetValue=0  RyPositionTargetValueUnits=deg  RyVelocityTargetSpecify=off  RyVelocityTargetPriority=High  RyVelocityTargetValue=0  RyVelocityTargetValueUnits=deg/s  RyEquilibriumPosition=0  RyEquilibriumPositionUnits=deg  RySpringStiffness=0  RySpringStiffnessUnits=N*m/deg  RyDampingCoefficient=0  RyDampingCoefficientUnits=N*m/(deg/s)  RyLowerLimitSpecify=off  RyLowerLimitBound=-90  RyLowerLimitBoundUnits=deg  RyLowerLimitStiffness=1e4  RyLowerLimitStiffnessUnits=N*m/deg  RyLowerLimitDamping=10  RyLowerLimitDampingUnits=N*m/(deg/s)  RyLowerLimitTransitionRegionWidth=0.1  RyLowerLimitTransitionRegionWidthUnits=deg  RyUpperLimitSpecify=off  RyUpperLimitBound=90  RyUpperLimitBoundUnits=deg  RyUpperLimitStiffness=1e4  RyUpperLimitStiffnessUnits=N*m/deg  RyUpperLimitDamping=10  RyUpperLimitDampingUnits=N*m/(deg/s)  RyUpperLimitTransitionRegionWidth=0.1  RyUpperLimitTransitionRegionWidthUnits=deg  RyTorqueActuationMode=NoTorque  RyMotionActuationMode=ComputedMotion  RySensePosition=off  RySenseVelocity=off  RySenseAcceleration=off  RySenseTorqueForce=off  RySenseLowerLimitTorqueForce=off  RySenseUpperLimitTorqueForce=off
  Universal Pushrod UA : sm_lib/Joints/Universal Joint  JointMode=Normal  CompositeWrenchDir=FollowerOnBase  CompositeWrenchFrame=FollowerFrame  SenseConstraintForce=off  SenseConstraintTorque=off  SenseTotalForce=off  SenseTotalTorque=off  RxPositionTargetSpecify=off  RxPositionTargetPriority=High  RxPositionTargetValue=0  RxPositionTargetValueUnits=deg  RxVelocityTargetSpecify=off  RxVelocityTargetPriority=High  RxVelocityTargetValue=0  RxVelocityTargetValueUnits=deg/s  RxEquilibriumPosition=0  RxEquilibriumPositionUnits=deg  RxSpringStiffness=0  RxSpringStiffnessUnits=N*m/deg  RxDampingCoefficient=0  RxDampingCoefficientUnits=N*m/(deg/s)  RxLowerLimitSpecify=off  RxLowerLimitBound=-90  RxLowerLimitBoundUnits=deg  RxLowerLimitStiffness=1e4  RxLowerLimitStiffnessUnits=N*m/deg  RxLowerLimitDamping=10  RxLowerLimitDampingUnits=N*m/(deg/s)  RxLowerLimitTransitionRegionWidth=0.1  RxLowerLimitTransitionRegionWidthUnits=deg  RxUpperLimitSpecify=off  RxUpperLimitBound=90  RxUpperLimitBoundUnits=deg  RxUpperLimitStiffness=1e4  RxUpperLimitStiffnessUnits=N*m/deg  RxUpperLimitDamping=10  RxUpperLimitDampingUnits=N*m/(deg/s)  RxUpperLimitTransitionRegionWidth=0.1  RxUpperLimitTransitionRegionWidthUnits=deg  RxTorqueActuationMode=NoTorque  RxMotionActuationMode=ComputedMotion  RxSensePosition=off  RxSenseVelocity=off  RxSenseAcceleration=off  RxSenseTorqueForce=off  RxSenseLowerLimitTorqueForce=off  RxSenseUpperLimitTorqueForce=off  RyPositionTargetSpecify=off  RyPositionTargetPriority=High  RyPositionTargetValue=0  RyPositionTargetValueUnits=deg  RyVelocityTargetSpecify=off  RyVelocityTargetPriority=High  RyVelocityTargetValue=0  RyVelocityTargetValueUnits=deg/s  RyEquilibriumPosition=0  RyEquilibriumPositionUnits=deg  RySpringStiffness=0  RySpringStiffnessUnits=N*m/deg  RyDampingCoefficient=0  RyDampingCoefficientUnits=N*m/(deg/s)  RyLowerLimitSpecify=off  RyLowerLimitBound=-90  RyLowerLimitBoundUnits=deg  RyLowerLimitStiffness=1e4  RyLowerLimitStiffnessUnits=N*m/deg  RyLowerLimitDamping=10  RyLowerLimitDampingUnits=N*m/(deg/s)  RyLowerLimitTransitionRegionWidth=0.1  RyLowerLimitTransitionRegionWidthUnits=deg  RyUpperLimitSpecify=off  RyUpperLimitBound=90  RyUpperLimitBoundUnits=deg  RyUpperLimitStiffness=1e4  RyUpperLimitStiffnessUnits=N*m/deg  RyUpperLimitDamping=10  RyUpperLimitDampingUnits=N*m/(deg/s)  RyUpperLimitTransitionRegionWidth=0.1  RyUpperLimitTransitionRegionWidthUnits=deg  RyTorqueActuationMode=NoTorque  RyMotionActuationMode=ComputedMotion  RySensePosition=off  RySenseVelocity=off  RySenseAcceleration=off  RySenseTorqueForce=off  RySenseLowerLimitTorqueForce=off  RySenseUpperLimitTorqueForce=off
  Universal Rack Rod : Subsystem
      mask Display: image('sm_car_variant_universal.png');
  Upper Arm : Subsystem  mask{popup_leftRight=Left, hp_in_f=hp_in_f_ua, hp_in_r=hp_in_r_ua, hp_out=hp_out_ua, ua_mass=ua_mass, clr_solid=Visual.UpperArm.clr, opc_solid=Visual.part.opc, rad_solid=Visual.UpperArm.rad}
      mask prompts: popup_leftRight "Left/Right"; hp_in_f "Inboard Front [xyz] (m)"; hp_in_r "Inboard Rear [xyz] (m)"; hp_out "Outboard [xyz] (m)"; ua_mass "Mass (kg)"; clr_solid "Color [RGB]"; opc_solid "Opacity (0-1)"; rad_solid "Radius (m)"
      mask init:
      | if(popup_leftRight == 1)
      |     rhs_susp = 1;
      | elseif(popup_leftRight == 2)
      |     rhs_susp = -1;
      | end
      | 
      | rhs_hp = [1 rhs_susp 1];
      | 
      |     hp_rod_f=hp_out-(hp_out-hp_in_f)/2;
      |     hp_rod_r=hp_out-(hp_out-hp_in_r)/2;
      mask TypeOptions popup_leftRight: Left | Right
      mask TypeOptions clr_solid: Arm F1/clr_solid | Arm F2/clr_solid | Arm R1/clr_solid | Arm R2/clr_solid
      mask TypeOptions opc_solid: Arm F1/opc_solid | Arm F2/opc_solid | Arm R1/opc_solid | Arm R2/opc_solid
      mask TypeOptions rad_solid: Arm F1/rad_solid | Arm F2/rad_solid | Arm R1/rad_solid | Arm R2/rad_solid
      mask DialogControl cont_ua Prompt: UA
      mask DialogControl cont_vis_ua Prompt: Visualization
      mask Display: image('sm_car_vehicle_linkage_dw_ua_IMAGE.png');
  UpperXYZ_m : nesl_utility/PS-Simulink Converter  PhysicalDomain=network_engine_domain  SubClassName=ps_output  LeftPortType=input  RightPortType=output  PseudoPeriodic=off  Frequencies=[]  VectorFormat=inherit  Unit=m  AffineConversion=off
  Upright : Subsystem  mask{popup_leftRight=Left, hp_ua_out=hp_out_ua, hp_la_out=hp_out_la, hp_upr_rod=hp_upr_rod, hp_upr_cg=hp_upr_cg, hp_upr_wc=hp_upr_wc, axle_len=axle_len, axle_whlc_to_bearing=axle_whlc_to_bearing, axle_mass=axle_mass, atoe=atoe, acamber=acamber, upr_mass=upr_mass, whl_init_spd_upr=whl_init_spd, clr_conn_upr=clr_conn_upr, opc_conn_upr=opc_conn_upr, size_conn_upr=size_conn_upr, clr_upr=clr_upr, opc_upr=opc_upr, radius_upr=radius_upr, clr_axle=clr_axle, opc_axle=opc_axle, radius_axle=radius_axle}
      mask prompts: popup_leftRight "Left/Right"; hp_ua_out "Upper Arm Outboard [xyz] (m)"; hp_la_out "Lower Arm Outboard [xyz] (m)"; hp_upr_rod "Track Rod Outboard [xyz] (m)"; hp_upr_cg "Center of Mass [xyz] (m)"; hp_upr_wc "Wheel Center [xyz] (m)"; axle_len "Axle Length (m)"; axle_whlc_to_bearing "Distance Wheel Ctr to Bearing (m)"; axle_mass "Axle Mass (kg)"; atoe "Toe Angle (deg)"; acamber "Camber Angle (deg)"; upr_mass "Upright Mass (kg)"; whl_init_spd_upr "Initial Wheel Speed (rad/s)"
      mask init:
      | % Set parameter for mirroring (+y or -y)
      | if(popup_leftRight == 1)
      |     rhs_upr = 1;
      | elseif(popup_leftRight == 2)
      |     rhs_upr = -1;
      | end
      | rhs_hp = [1 rhs_upr 1];
      | 
      | % Additional hardpoint at center of upright
      | % Used as attachment points for axle and steering arm
      | hp_upr_ctr = (hp_ua_out+hp_la_out)/2;
      mask TypeOptions popup_leftRight: Left | Right
      mask TypeOptions axle_mass: Axle/Mass
      mask TypeOptions upr_mass:
      | Inertia
      | CG/Mass
      mask TypeOptions whl_init_spd_upr: Revolute/whl_init_spd_jnt
      mask TypeOptions clr_conn_upr:
      | Vis Upright LA/GraphicDiffuseColor | Vis Upright UA/GraphicDiffuseColor | Vis Wheel
      | Center/GraphicDiffuseColor
      mask TypeOptions opc_conn_upr:
      | Vis Upright LA/GraphicOpacity | Vis Upright UA/GraphicOpacity | Vis Wheel
      | Center/GraphicOpacity
      mask TypeOptions clr_upr:
      | Upright/clr_solid | Steering Arm/clr_solid | Bearing
      | Carrier/GraphicDiffuseColor
      mask TypeOptions opc_upr: Upright/opc_solid | Steering Arm/opc_solid
      mask TypeOptions radius_upr: Upright/rad_solid | Steering Arm/rad_solid
      mask TypeOptions clr_axle: Axle/GraphicDiffuseColor
      mask TypeOptions opc_axle: Axle/GraphicOpacity
      mask TypeOptions radius_axle: Axle/CylinderRadius
      mask DialogControl cont_upright Prompt: Upright
      mask DialogControl grp_init Prompt: Initialization
      mask DialogControl cont_vis_upr Prompt: Visualization
      mask DialogControl text_clr_upr Prompt: Color [RGB]
      mask DialogControl text_opc_upr Prompt: Opac. (0-1)
      mask DialogControl text_size_upr Prompt: Size (m)
      mask DialogControl text_conn_upr Prompt: Connections
      mask DialogControl text_upright Prompt: Upright
      mask DialogControl text_stub_axle Prompt: Axle
      mask Display: image('sm_car_vehicle_linkage_dw_upr_IMAGE.png');
  Rack : PMIOPort  Side=Right
  Ref : PMIOPort  Port=2  Side=Right
  WhlC : PMIOPort  Port=3  Side=Left
  RaceSpin : PMIOPort  Port=4  Side=Left
  RaceFix : PMIOPort  Port=5  Side=Left
  Axle1D : PMIOPort  Port=6  Side=Left
  AxleIn : PMIOPort  Port=7  Side=Left
  S : PMIOPort  Port=8  Side=Left
  D : PMIOPort  Port=9  Side=Left
  LAo : PMIOPort  Port=10  Side=Left
  Out Bus Element : Outport  VectorParamsAs1DForOutWhenUnconnected=off  PortName=m  Element=Shock
  Out Bus Element1 : Outport  VectorParamsAs1DForOutWhenUnconnected=off  PortName=m  Element=Upright
  Out Bus Element2 : Outport  VectorParamsAs1DForOutWhenUnconnected=off  PortName=m  Element=BushLA
  Out Bus Element3 : Outport  VectorParamsAs1DForOutWhenUnconnected=off  PortName=m  Element=BushUA
  Out Bus Element4 : Outport  VectorParamsAs1DForOutWhenUnconnected=off  PortName=m  Element=UprUA_F
  Out Bus Element5 : Outport  VectorParamsAs1DForOutWhenUnconnected=off  PortName=m  Element=UprLA_F
  Out Bus Element11 : Outport  VectorParamsAs1DForOutWhenUnconnected=off  PortName=m  Element=UA_F
  Out Bus Element6 : Outport  VectorParamsAs1DForOutWhenUnconnected=off  PortName=m  Element=LA_F
  Out Bus Element7 : Outport  VectorParamsAs1DForOutWhenUnconnected=off  PortName=m  Element=Push_F
  Out Bus Element8 : Outport  VectorParamsAs1DForOutWhenUnconnected=off  PortName=m  Element=TrackRod_F
  Out Bus Element9 : Outport  VectorParamsAs1DForOutWhenUnconnected=off  PortName=m  Element=UprTrack-F
  UpperUprightXYZ : Outport  VectorParamsAs1DForOutWhenUnconnected=off  PortName=m  Element=UpperUprightXYZ
  LowerUprightXYZ : Outport  VectorParamsAs1DForOutWhenUnconnected=off  PortName=m  Element=LowerUprightXYZ
  wires:
  Upright/1(m) -> Out Bus Element1/1
  Shock/1 -> Out Bus Element/1
  HP LA/1 -> Out Bus Element2/1
  HP UA/1 -> Out Bus Element3/1
  PS-Simulink Converter/1 -> Out Bus Element4/1
  PS-Simulink Converter1/1 -> Out Bus Element5/1
  Upper Arm/1(m) -> Out Bus Element11/1
  Lower Arm/1(m) -> Out Bus Element6/1
  Push Rod/1(m) -> Out Bus Element7/1
  Track Rod/1(m) -> Out Bus Element8/1
  PS-Simulink Converter2/1 -> Out Bus Element9/1
  UpperXYZ_m/1 -> UpperUprightXYZ/1
  LowerXYZ_m/1 -> LowerUprightXYZ/1
  connections:
  Universal Pushrod UA/RConn1 -- Lower Arm/LConn1
  AxleIn/RConn1 -- Upright/LConn5
  RaceFix/RConn1 -- Upright/LConn3
  RaceSpin/RConn1 -- Upright/LConn2
  Shock/RConn2 -- Universal HP Spring/RConn1
  Upright/LConn1 -- WhlC/RConn1
  Ref/RConn1 -- Hardpoints/RConn1 -- Transform Sensor/LConn1 -- Transform Sensor1/LConn1
  HP UA/LConn1 -- Hardpoints/LConn1
  Spherical Rod Upright/RConn1 -- Upright/RConn1
  Rack/RConn1 -- Transform Track Rod Inboard/LConn1
  Upright/LConn4 -- Axle1D/RConn1
  HP UA/RConn1 -- Upper Arm/RConn1
  HP LA/LConn1 -- Hardpoints/LConn4
  Spherical LA Upright/RConn1 -- Upright/RConn3 -- Transform Sensor1/RConn1
  Spherical UA Upright/LConn1 -- Upper Arm/LConn1
  HP LA/RConn1 -- Lower Arm/RConn1
  Spherical LA Upright/LConn1 -- Lower Arm/LConn2
  Spherical UA Upright/RConn1 -- Upright/RConn2 -- Transform Sensor/RConn1
  Spherical Rod Upright/LConn1 -- Track Rod/LConn1
  Universal Rack Rod/LConn1 -- Track Rod/RConn1
  Universal Rack Rod/RConn1 -- Transform Track Rod Inboard/RConn1
  Transform Ref Arb/LConn1 -- LAo/RConn1
  D/RConn1 -- Shock/RConn1 -- S/RConn1
  HP Bellcrank/RConn1 -- Bellcrank/RConn1
  Transform Ref Arb/RConn1 -- Bellcrank/LConn2
  Universal Pushrod UA/LConn1 -- Push Rod/LConn1
  Spherical Pushrod Bellcrank/RConn1 -- Bellcrank/LConn1
  Spherical Pushrod Bellcrank/LConn1 -- Push Rod/RConn1
  HP Bellcrank/LConn1 -- Hardpoints/LConn2
  Shock/LConn1 -- Spherical Bellcrank Shock/RConn1
  Universal HP Spring/LConn1 -- Hardpoints/LConn3
  Spherical Bellcrank Shock/LConn1 -- Bellcrank/LConn3
  PS-Simulink Converter/LConn1 -- Spherical UA Upright/RConn2
  PS-Simulink Converter1/LConn1 -- Spherical LA Upright/RConn2
  Spherical Rod Upright/RConn2 -- PS-Simulink Converter2/LConn1
  Transform Sensor/RConn2 -- UpperXYZ_m/LConn1
  Transform Sensor1/RConn2 -- LowerXYZ_m/LConn1

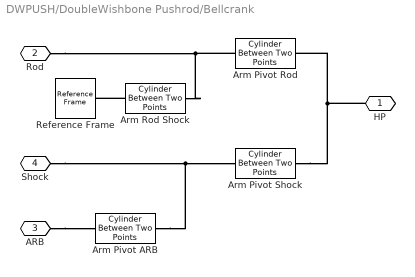
== system DWPUSH/DoubleWishbone Pushrod/Bellcrank ==
  Arm Pivot ARB : Suspension_Utilities/Cylinder Between Two Points  hp_b=hp_bcr_shock.*rhs_hp  hp_f=hp_arb.*rhs_hp  Mass=bcr_mass*0.001  clr_solid=clr_bcr  opc_solid=opc_bcr  rad_solid=radius_bcr
      settings: SourceProductName=SmCar - Suspension Utilites
  Arm Pivot Rod : Suspension_Utilities/Cylinder Between Two Points  hp_b=hp_bcr_pivot.*rhs_hp  hp_f=hp_rod.*rhs_hp  Mass=bcr_mass/3  clr_solid=clr_bcr  opc_solid=opc_bcr  rad_solid=radius_bcr
      settings: SourceProductName=SmCar - Suspension Utilites
  Arm Pivot Shock : Suspension_Utilities/Cylinder Between Two Points  hp_b=hp_bcr_pivot.*rhs_hp  hp_f=hp_bcr_shock.*rhs_hp  Mass=bcr_mass/3  clr_solid=clr_bcr  opc_solid=opc_bcr  rad_solid=radius_bcr
      settings: SourceProductName=SmCar - Suspension Utilites
  Arm Rod Shock : Suspension_Utilities/Cylinder Between Two Points  hp_b=hp_rod.*rhs_hp  hp_f=hp_bcr_shock.*rhs_hp  Mass=bcr_mass/3  clr_solid=clr_bcr  opc_solid=opc_bcr  rad_solid=radius_bcr
      settings: SourceProductName=SmCar - Suspension Utilites
  Reference Frame : sm_lib/Frames and Transforms/Reference Frame
  HP : PMIOPort  Side=Right
  Rod : PMIOPort  Port=2  Side=Left
  ARB : PMIOPort  Port=3  Side=Left
  Shock : PMIOPort  Port=4  Side=Left
  connections:
  Arm Rod Shock/RConn1 -- Reference Frame/RConn1
  Shock/RConn1 -- Arm Pivot ARB/LConn1 -- Arm Pivot Shock/RConn1
  HP/RConn1 -- Arm Pivot Rod/LConn1 -- Arm Pivot Shock/LConn1
  Rod/RConn1 -- Arm Pivot Rod/RConn1 -- Arm Rod Shock/LConn1
  ARB/RConn1 -- Arm Pivot ARB/RConn1
